simulink model "simulink"  (R2024b)
settings: Solver=ode15s  StartTime=0.0  StopTime=.3  RelTol=1e-3
values from neighbouring files (symbols this model uses):
  B_m = (kfi^2 * I_anl) / (V_an - R_a * I_anl)    (= 5.06615156069e-07)    [code.m]
  Jm = 5.05e-7    (= 5.05e-07)    [code.m]
  kfi = 9.18e-3    (= 0.00918)    [code.m]
  ki = 1/tc    (= 32.7207920792)    [code.m]
  kp = (tau_m+tau_e)/(tc+ tau_e)    (= 0.201485710943)    [code.m]
  L_a = 0.058e-3    (= 5.8e-05)    [code.m]
  R_a = 1.02    [code.m]
  ref_rpm = 10700    [code.m]
  T_n = 14.6e-3    (= 0.0146)    [code.m]
  tau_e = L_a / R_a    (= 5.6862745098e-05)    [code.m]
  tau_m = (Jm * R_a) / (kfi^2)    (= 0.0061123214718)    [code.m]
  V_an = 12    [code.m]
libraries: slpidlib x4, spsControlledVoltageSourceLib x2, spsDCMachineLib x2, sps_lib x1
settings Model: Creator=Compu City  LastModifiedBy=Compu City
settings SolverCC: MaxConsecutiveMinStep=5

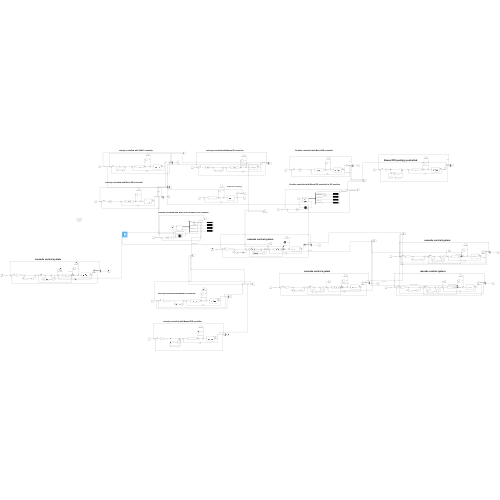
[thumbnail: Simulink's stored preview of the top-level diagram]
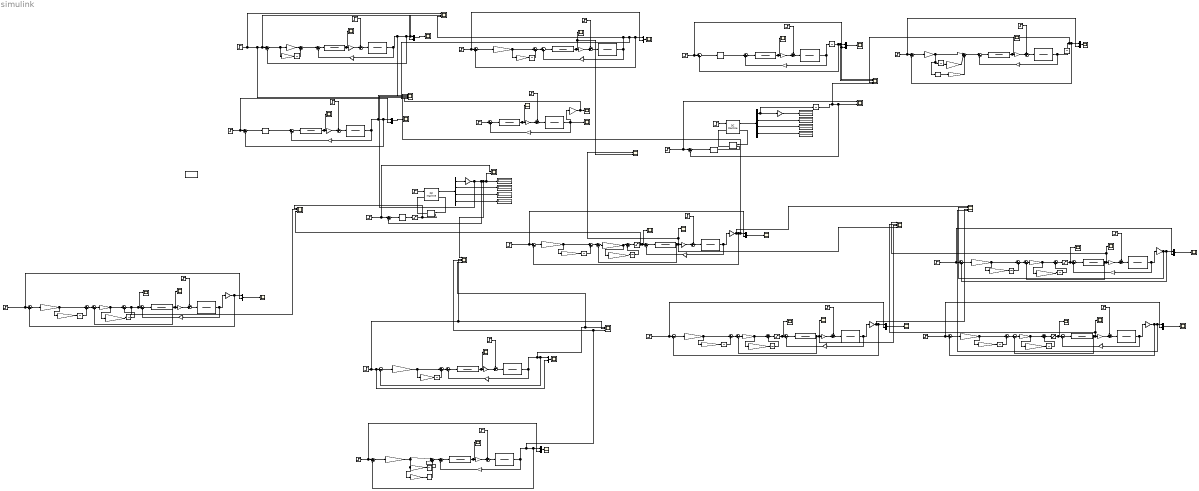
== system simulink ==
  note: Without Any controlling
  note: Manual PID position controlled
  note: velocity controlled with Manual PI controller
  note: velocity controlled with ICM PI controller
  note: velocity controlled with Block PID controller
  note: velocity controlled with Block PID controller in DC machine
  note: Position controlled with Block PID controller in DC machine
  note: Position controlled with Block PID controller
  note: cascade control system
  note: velocity controlled with Manual PI controller
  note: velocity controlled with Manual PID controller
  note: cascade control system
  note: cascade control system
  note: cascade control system
  note: cascade control system
  Bus Selector1 : BusSelector  OutputSignals=Speed wm (rad/s),Armature current ia (A),Field current if (A),Electrical torque Te (n m)
  Bus Selector2 : BusSelector  OutputSignals=Speed wm (rad/s),Armature current ia (A),Field current if (A),Electrical torque Te (n m)
  Controlled Voltage Source : spsControlledVoltageSourceLib/Controlled Voltage Source  Initialize=on  Source_Type=AC  Amplitude=0  Phase=0  Frequency=0  Measurements=None
  Controlled Voltage Source1 : spsControlledVoltageSourceLib/Controlled Voltage Source  Initialize=on  Source_Type=AC  Amplitude=0  Phase=0  Frequency=0  Measurements=None
  Current comparison : Scope  NumInputPorts=2
  DC permanent magnetic motor1 : spsDCMachineLib/DC Machine  PresetModel=No  MechanicalLoad=Torque TL  FieldType=Permanent magnet  ShowDetailedParameters=on  MeasurementBus=off  RLa=[1.02 5.8*10^-5]  RLf=[180 71.47]  Laf=1.345  MachineConstant=Torque constant (N.m/A)  Ke=1.8  Kt=kfi  J=Jm  Bm=B_m  Tf=0  w0=0  Ifinit=1  TsPowergui=0  TsBlock=-1
  DC permanent magnetic motor2 : spsDCMachineLib/DC Machine  PresetModel=No  MechanicalLoad=Torque TL  FieldType=Permanent magnet  ShowDetailedParameters=on  MeasurementBus=off  RLa=[1.02 5.8*10^-5]  RLf=[180 71.47]  Laf=1.345  MachineConstant=Torque constant (N.m/A)  Ke=1.8  Kt=kfi  J=Jm  Bm=B_m  Tf=0  w0=0  Ifinit=1  TsPowergui=0  TsBlock=-1
  Derivative : Derivative
  Derivative3 : Derivative
  Display{1..4,8..11} (8 alike) : Display
  External load{1..13} (13 alike) : Step  Time=0.02  After=T_n  SampleTime=0
  Gain : Gain  Gain=tau_e*60
  Gain1 : Gain  Gain=1/tau_m
  Gain{2,4..6,9..12,14..15,17..18,21,23,27..28,33,36..37,41..42,44,49..50,54..55} (26 alike) : Gain  Gain=kfi
  Gain{13,26,34..35,40,48} (6 alike) : Gain  Gain=1/(tau_m)
  Gain16 : Gain  Gain=30/pi
  Gain{8,19,45,51,56} (5 alike) : Gain  Gain=0.00705
  Gain20 : Gain  Gain=1/(tau_m*5)
  Gain22 : Gain  Gain=1/(tau_m/1000)
  Gain{24,47,53,58} (4 alike) : Gain  Gain=0.000705
  Gain25 : Gain  Gain=kp*10
  Gain29 : Gain  Gain=0.005
  Gain3 : Gain  Gain=ki
  Gain30 : Gain  Gain=1/(tau_m/1000)
  Gain31 : Gain  Gain=0.005
  Gain32 : Gain  Gain=1/(tau_m/10000)
  Gain38 : Gain  Gain=0.05
  Gain39 : Gain  Gain=tau_e
  Gain43 : Gain  Gain=0.05
  Gain46 : Gain  Gain=1/(tau_m/10000)
  Gain52 : Gain  Gain=1/(tau_m/10)
  Gain57 : Gain  Gain=1/(tau_m/1000)
  Gain7 : Gain  Gain=kp
  I{,1..5,8..9} (8 alike) : Scope
  Integrator{,1..17} (18 alike) : Integrator
  Mux{1..12} (12 alike) : Mux  Inputs=2
  PID Controller : slpidlib/PID Controller  Controller=PID  Form=Parallel  TimeDomain=Continuous-time  UseExternalTs=off  SampleTime=-1  IntegratorMethod=Forward Euler  FilterMethod=Forward Euler  ControllerParametersSource=internal  P=0.0119953669001722  I=2.21317544504697  UseKiTs=off  D=3.8924087618185e-06  UseExternalDerivativeSource=off  N=383.757391684538  UseFilter=on  TunerSelectOption=Transfer Function Based (PID Tuner App)  InitialConditionSource=internal  InitialConditionForIntegrator=0  InitialConditionForFilter=0  DifferentiatorICPrevScaledInput=0  ExternalReset=none  TrackingMode=off  Kt=1  LimitOutput=off  SatLimitsSource=internal  UpperSaturationLimit=inf  LowerSaturationLimit=-inf  LinearizeAsGain=on  AntiWindupMode=none  Kb=1  LimitIntegrator=off  UpperIntegratorSaturationLimit=inf  LowerIntegratorSaturationLimit=-inf  POutMin=[]  POutMax=[]  IOutMin=[]  IOutMax=[]  DOutMin=[]  DOutMax=[]  NOutMin=[]  NOutMax=[]  SumOutMin=[]  SumOutMax=[]  SaturationOutMin=[]  SaturationOutMax=[]  PParamMin=[]  PParamMax=[]  IParamMin=[]  IParamMax=[]  DParamMin=[]  DParamMax=[]  NParamMin=[]  NParamMax=[]  KbParamMin=[]  KbParamMax=[]  KtParamMin=[]  KtParamMax=[]  KbOutMin=[]  KbOutMax=[]  KtOutMin=[]  KtOutMax=[]  IntegratorOutMin=[]  IntegratorOutMax=[]  FilterOutMin=[]  FilterOutMax=[]  SumI1OutMin=[]  SumI1OutMax=[]  SumI2OutMin=[]  SumI2OutMax=[]  SumI3OutMin=[]  SumI3OutMax=[]  SumI4OutMin=[]  SumI4OutMax=[]  SumDOutMin=[]  SumDOutMax=[]  DifferentiatorOutMin=[]  DifferentiatorOutMax=[]  FilterDiffOutCoefMin=[]  FilterDiffOutCoefMax=[]  ReciprocalOutMin=[]  ReciprocalOutMax=[]  SumDenOutMin=[]  SumDenOutMax=[]  SumNumOutMin=[]  SumNumOutMax=[]  DivideOutMin=[]  DivideOutMax=[]  UdiffTsProdOutMin=[]  UdiffTsProdOutMax=[]  NTsProdOutMin=[]  NTsProdOutMax=[]  UintegralTsProdOutMin=[]  UintegralTsProdOutMax=[]  UngainTsProdOutMin=[]  UngainTsProdOutMax=[]  ClampingZeroOutDataTypeStr=Inherit: Inherit via back propagation  ClampingZeroOutMin=[]  ClampingZeroOutMax=[]  FilterDenConstantOutDataTypeStr=Inherit: Inherit via back propagation  FilterDenConstantOutMin=[]  FilterDenConstantOutMax=[]  PCopyOutDataTypeStr=Inherit: Inherit via back propagation  PCopyOutMin=[]  PCopyOutMax=[]  NCopyOutDataTypeStr=Inherit: Inherit via back propagation  NCopyOutMin=[]  NCopyOutMax=[]  IntegratorContinuousStateAttributes=''  IntegratorStateMustResolveToSignalObject=off  IntegratorRTWStateStorageClass=Auto  FilterContinuousStateAttributes=''  FilterStateMustResolveToSignalObject=off  FilterRTWStateStorageClass=Auto  ParallelPVariant=InternalParameters  IdealPVariant=Disabled  IVariant=InternalParameters  DVariant=InternalParameters  IntegratorVariant=Continuous  SatVariant=Disabled  AWVariant=Passthrough  PCopyVariant=Disabled  TRVariant=Disabled  FdbkBlocksVariant=Forward  IdealPFdbkVariant=Disabled  SatFdbkVariant=Disabled  DerivativeFilterVariant=ContFilter  NVariant=InternalParameters  NCopyVariant=Disabled  FilterICVariant=InternalICsFilter  IntegratorICVariant=InternalICs  ExternalResetVariant=Disabled  TRSumVariant=Passthrough  SumFdbkVariant=Disabled  SumVariant=Sum_PID  TsampFilterVariant=InternalTs  TsampNgainVariant=Passthrough  TsampIntegralVariant=Disabled_SignalSpec  ExternalSaturationOutDataTypeStr=Inherit: Same as second input  DerivativeSourceVariant=ErrorSignal  PreIntVariant=InternalPreInt
  PID Controller1 : slpidlib/PID Controller  Controller=PID  Form=Parallel  TimeDomain=Continuous-time  UseExternalTs=off  SampleTime=-1  IntegratorMethod=Forward Euler  FilterMethod=Forward Euler  ControllerParametersSource=internal  P=0.00135864322894718  I=0.306131273508745  UseKiTs=off  D=4.02045915696409e-07  UseExternalDerivativeSource=off  N=693.137788969892  UseFilter=on  TunerSelectOption=Transfer Function Based (PID Tuner App)  InitialConditionSource=internal  InitialConditionForIntegrator=0  InitialConditionForFilter=0  DifferentiatorICPrevScaledInput=0  ExternalReset=none  TrackingMode=off  Kt=1  LimitOutput=off  SatLimitsSource=internal  UpperSaturationLimit=inf  LowerSaturationLimit=-inf  LinearizeAsGain=on  AntiWindupMode=none  Kb=1  LimitIntegrator=off  UpperIntegratorSaturationLimit=inf  LowerIntegratorSaturationLimit=-inf  POutMin=[]  POutMax=[]  IOutMin=[]  IOutMax=[]  DOutMin=[]  DOutMax=[]  NOutMin=[]  NOutMax=[]  SumOutMin=[]  SumOutMax=[]  SaturationOutMin=[]  SaturationOutMax=[]  PParamMin=[]  PParamMax=[]  IParamMin=[]  IParamMax=[]  DParamMin=[]  DParamMax=[]  NParamMin=[]  NParamMax=[]  KbParamMin=[]  KbParamMax=[]  KtParamMin=[]  KtParamMax=[]  KbOutMin=[]  KbOutMax=[]  KtOutMin=[]  KtOutMax=[]  IntegratorOutMin=[]  IntegratorOutMax=[]  FilterOutMin=[]  FilterOutMax=[]  SumI1OutMin=[]  SumI1OutMax=[]  SumI2OutMin=[]  SumI2OutMax=[]  SumI3OutMin=[]  SumI3OutMax=[]  SumI4OutMin=[]  SumI4OutMax=[]  SumDOutMin=[]  SumDOutMax=[]  DifferentiatorOutMin=[]  DifferentiatorOutMax=[]  FilterDiffOutCoefMin=[]  FilterDiffOutCoefMax=[]  ReciprocalOutMin=[]  ReciprocalOutMax=[]  SumDenOutMin=[]  SumDenOutMax=[]  SumNumOutMin=[]  SumNumOutMax=[]  DivideOutMin=[]  DivideOutMax=[]  UdiffTsProdOutMin=[]  UdiffTsProdOutMax=[]  NTsProdOutMin=[]  NTsProdOutMax=[]  UintegralTsProdOutMin=[]  UintegralTsProdOutMax=[]  UngainTsProdOutMin=[]  UngainTsProdOutMax=[]  ClampingZeroOutDataTypeStr=Inherit: Inherit via back propagation  ClampingZeroOutMin=[]  ClampingZeroOutMax=[]  FilterDenConstantOutDataTypeStr=Inherit: Inherit via back propagation  FilterDenConstantOutMin=[]  FilterDenConstantOutMax=[]  PCopyOutDataTypeStr=Inherit: Inherit via back propagation  PCopyOutMin=[]  PCopyOutMax=[]  NCopyOutDataTypeStr=Inherit: Inherit via back propagation  NCopyOutMin=[]  NCopyOutMax=[]  IntegratorContinuousStateAttributes=''  IntegratorStateMustResolveToSignalObject=off  IntegratorRTWStateStorageClass=Auto  FilterContinuousStateAttributes=''  FilterStateMustResolveToSignalObject=off  FilterRTWStateStorageClass=Auto  ParallelPVariant=InternalParameters  IdealPVariant=Disabled  IVariant=InternalParameters  DVariant=InternalParameters  IntegratorVariant=Continuous  SatVariant=Disabled  AWVariant=Passthrough  PCopyVariant=Disabled  TRVariant=Disabled  FdbkBlocksVariant=Forward  IdealPFdbkVariant=Disabled  SatFdbkVariant=Disabled  DerivativeFilterVariant=ContFilter  NVariant=InternalParameters  NCopyVariant=Disabled  FilterICVariant=InternalICsFilter  IntegratorICVariant=InternalICs  ExternalResetVariant=Disabled  TRSumVariant=Passthrough  SumFdbkVariant=Disabled  SumVariant=Sum_PID  TsampFilterVariant=InternalTs  TsampNgainVariant=Passthrough  TsampIntegralVariant=Disabled_SignalSpec  ExternalSaturationOutDataTypeStr=Inherit: Same as second input  DerivativeSourceVariant=ErrorSignal  PreIntVariant=InternalPreInt
  PID Controller2 : slpidlib/PID Controller  Controller=PID  Form=Parallel  TimeDomain=Continuous-time  UseExternalTs=off  SampleTime=-1  IntegratorMethod=Forward Euler  FilterMethod=Forward Euler  ControllerParametersSource=internal  P=8.0055285463139  I=469.188134848807  UseKiTs=off  D=0.034037625993495  UseExternalDerivativeSource=off  N=70209.7443182031  UseFilter=on  TunerSelectOption=Transfer Function Based (PID Tuner App)  InitialConditionSource=internal  InitialConditionForIntegrator=0  InitialConditionForFilter=0  DifferentiatorICPrevScaledInput=0  ExternalReset=none  TrackingMode=off  Kt=1  LimitOutput=off  SatLimitsSource=internal  UpperSaturationLimit=inf  LowerSaturationLimit=-inf  LinearizeAsGain=on  AntiWindupMode=none  Kb=1  LimitIntegrator=off  UpperIntegratorSaturationLimit=inf  LowerIntegratorSaturationLimit=-inf  POutMin=[]  POutMax=[]  IOutMin=[]  IOutMax=[]  DOutMin=[]  DOutMax=[]  NOutMin=[]  NOutMax=[]  SumOutMin=[]  SumOutMax=[]  SaturationOutMin=[]  SaturationOutMax=[]  PParamMin=[]  PParamMax=[]  IParamMin=[]  IParamMax=[]  DParamMin=[]  DParamMax=[]  NParamMin=[]  NParamMax=[]  KbParamMin=[]  KbParamMax=[]  KtParamMin=[]  KtParamMax=[]  KbOutMin=[]  KbOutMax=[]  KtOutMin=[]  KtOutMax=[]  IntegratorOutMin=[]  IntegratorOutMax=[]  FilterOutMin=[]  FilterOutMax=[]  SumI1OutMin=[]  SumI1OutMax=[]  SumI2OutMin=[]  SumI2OutMax=[]  SumI3OutMin=[]  SumI3OutMax=[]  SumI4OutMin=[]  SumI4OutMax=[]  SumDOutMin=[]  SumDOutMax=[]  DifferentiatorOutMin=[]  DifferentiatorOutMax=[]  FilterDiffOutCoefMin=[]  FilterDiffOutCoefMax=[]  ReciprocalOutMin=[]  ReciprocalOutMax=[]  SumDenOutMin=[]  SumDenOutMax=[]  SumNumOutMin=[]  SumNumOutMax=[]  DivideOutMin=[]  DivideOutMax=[]  UdiffTsProdOutMin=[]  UdiffTsProdOutMax=[]  NTsProdOutMin=[]  NTsProdOutMax=[]  UintegralTsProdOutMin=[]  UintegralTsProdOutMax=[]  UngainTsProdOutMin=[]  UngainTsProdOutMax=[]  ClampingZeroOutDataTypeStr=Inherit: Inherit via back propagation  ClampingZeroOutMin=[]  ClampingZeroOutMax=[]  FilterDenConstantOutDataTypeStr=Inherit: Inherit via back propagation  FilterDenConstantOutMin=[]  FilterDenConstantOutMax=[]  PCopyOutDataTypeStr=Inherit: Inherit via back propagation  PCopyOutMin=[]  PCopyOutMax=[]  NCopyOutDataTypeStr=Inherit: Inherit via back propagation  NCopyOutMin=[]  NCopyOutMax=[]  IntegratorContinuousStateAttributes=''  IntegratorStateMustResolveToSignalObject=off  IntegratorRTWStateStorageClass=Auto  FilterContinuousStateAttributes=''  FilterStateMustResolveToSignalObject=off  FilterRTWStateStorageClass=Auto  ParallelPVariant=InternalParameters  IdealPVariant=Disabled  IVariant=InternalParameters  DVariant=InternalParameters  IntegratorVariant=Continuous  SatVariant=Disabled  AWVariant=Passthrough  PCopyVariant=Disabled  TRVariant=Disabled  FdbkBlocksVariant=Forward  IdealPFdbkVariant=Disabled  SatFdbkVariant=Disabled  DerivativeFilterVariant=ContFilter  NVariant=InternalParameters  NCopyVariant=Disabled  FilterICVariant=InternalICsFilter  IntegratorICVariant=InternalICs  ExternalResetVariant=Disabled  TRSumVariant=Passthrough  SumFdbkVariant=Disabled  SumVariant=Sum_PID  TsampFilterVariant=InternalTs  TsampNgainVariant=Passthrough  TsampIntegralVariant=Disabled_SignalSpec  ExternalSaturationOutDataTypeStr=Inherit: Same as second input  DerivativeSourceVariant=ErrorSignal  PreIntVariant=InternalPreInt
  PID Controller3 : slpidlib/PID Controller  Controller=PID  Form=Parallel  TimeDomain=Continuous-time  UseExternalTs=off  SampleTime=-1  IntegratorMethod=Forward Euler  FilterMethod=Forward Euler  ControllerParametersSource=internal  P=16.6827824255638  I=704.189736175567  UseKiTs=off  D=0.0978151293443874  UseExternalDerivativeSource=off  N=92341.2012278854  UseFilter=on  TunerSelectOption=Transfer Function Based (PID Tuner App)  InitialConditionSource=internal  InitialConditionForIntegrator=0  InitialConditionForFilter=0  DifferentiatorICPrevScaledInput=0  ExternalReset=none  TrackingMode=off  Kt=1  LimitOutput=off  SatLimitsSource=internal  UpperSaturationLimit=inf  LowerSaturationLimit=-inf  LinearizeAsGain=on  AntiWindupMode=none  Kb=1  LimitIntegrator=off  UpperIntegratorSaturationLimit=inf  LowerIntegratorSaturationLimit=-inf  POutMin=[]  POutMax=[]  IOutMin=[]  IOutMax=[]  DOutMin=[]  DOutMax=[]  NOutMin=[]  NOutMax=[]  SumOutMin=[]  SumOutMax=[]  SaturationOutMin=[]  SaturationOutMax=[]  PParamMin=[]  PParamMax=[]  IParamMin=[]  IParamMax=[]  DParamMin=[]  DParamMax=[]  NParamMin=[]  NParamMax=[]  KbParamMin=[]  KbParamMax=[]  KtParamMin=[]  KtParamMax=[]  KbOutMin=[]  KbOutMax=[]  KtOutMin=[]  KtOutMax=[]  IntegratorOutMin=[]  IntegratorOutMax=[]  FilterOutMin=[]  FilterOutMax=[]  SumI1OutMin=[]  SumI1OutMax=[]  SumI2OutMin=[]  SumI2OutMax=[]  SumI3OutMin=[]  SumI3OutMax=[]  SumI4OutMin=[]  SumI4OutMax=[]  SumDOutMin=[]  SumDOutMax=[]  DifferentiatorOutMin=[]  DifferentiatorOutMax=[]  FilterDiffOutCoefMin=[]  FilterDiffOutCoefMax=[]  ReciprocalOutMin=[]  ReciprocalOutMax=[]  SumDenOutMin=[]  SumDenOutMax=[]  SumNumOutMin=[]  SumNumOutMax=[]  DivideOutMin=[]  DivideOutMax=[]  UdiffTsProdOutMin=[]  UdiffTsProdOutMax=[]  NTsProdOutMin=[]  NTsProdOutMax=[]  UintegralTsProdOutMin=[]  UintegralTsProdOutMax=[]  UngainTsProdOutMin=[]  UngainTsProdOutMax=[]  ClampingZeroOutDataTypeStr=Inherit: Inherit via back propagation  ClampingZeroOutMin=[]  ClampingZeroOutMax=[]  FilterDenConstantOutDataTypeStr=Inherit: Inherit via back propagation  FilterDenConstantOutMin=[]  FilterDenConstantOutMax=[]  PCopyOutDataTypeStr=Inherit: Inherit via back propagation  PCopyOutMin=[]  PCopyOutMax=[]  NCopyOutDataTypeStr=Inherit: Inherit via back propagation  NCopyOutMin=[]  NCopyOutMax=[]  IntegratorContinuousStateAttributes=''  IntegratorStateMustResolveToSignalObject=off  IntegratorRTWStateStorageClass=Auto  FilterContinuousStateAttributes=''  FilterStateMustResolveToSignalObject=off  FilterRTWStateStorageClass=Auto  ParallelPVariant=InternalParameters  IdealPVariant=Disabled  IVariant=InternalParameters  DVariant=InternalParameters  IntegratorVariant=Continuous  SatVariant=Disabled  AWVariant=Passthrough  PCopyVariant=Disabled  TRVariant=Disabled  FdbkBlocksVariant=Forward  IdealPFdbkVariant=Disabled  SatFdbkVariant=Disabled  DerivativeFilterVariant=ContFilter  NVariant=InternalParameters  NCopyVariant=Disabled  FilterICVariant=InternalICsFilter  IntegratorICVariant=InternalICs  ExternalResetVariant=Disabled  TRSumVariant=Passthrough  SumFdbkVariant=Disabled  SumVariant=Sum_PID  TsampFilterVariant=InternalTs  TsampNgainVariant=Passthrough  TsampIntegralVariant=Disabled_SignalSpec  ExternalSaturationOutDataTypeStr=Inherit: Same as second input  DerivativeSourceVariant=ErrorSignal  PreIntVariant=InternalPreInt
  Saturation{1..3,5..6} (5 alike) : Saturate  UpperLimit=V_an  LowerLimit=-V_an
  Scope{,5,7,9..10} (5 alike) : Scope
  Scope1 : Scope  NumInputPorts=3
  Scope11 : Scope  NumInputPorts=3
  Scope{6,8,12,14} (4 alike) : Scope  NumInputPorts=4
  Scope13 : Scope  NumInputPorts=3
  Scope2 : Scope  NumInputPorts=2
  Scope3 : Scope  NumInputPorts=7
  Scope4 : Scope  NumInputPorts=2
  Sum{,1..2,5,7..9,11,13,16..18,21..23,27..28,31..32,34,37..38,41..42,45..46,48,51..52,54,57..58} (32 alike) : Sum  Inputs=|+-
  Sum{3,10,12,14..15,19,25,29,35,39,43,49,55} (13 alike) : Sum  Inputs=-+|
  Sum{4,6,20,24,30,33,36,44,47,50,53,56,59} (13 alike) : Sum  Inputs=|++
  Sum26 : Sum  Inputs=|+++
  Sum40 : Sum  Inputs=|+++
  T_N : Step  Time=0.02  After=T_n  SampleTime=0
  T_N1 : Step  Time=0.02  After=T_n  SampleTime=0
  Transfer Fcn{1..2,5,7,9,11,13,15,17,19,21,23,25} (13 alike) : TransferFcn  Denominator=[ L_a R_a]
  Transfer Fcn{3..4,6,8,10,12,14,16,18,20,22,24,26} (13 alike) : TransferFcn  Denominator=[ Jm B_m ]
  U(S){1..2,4,6,8..13} (10 alike) : Step  Time=0.02  After=ref_rpm  SampleTime=0
  U(S)3 : Step  Time=0.02  After=V_an  SampleTime=0
  U(S)5 : Step  Time=0.02  After=pi  SampleTime=0
  U(S)7 : Step  Time=0.02  After=pi  SampleTime=0
  U(t)1 : Step  Time=0.02  After=pi  SampleTime=0
  U(t)2 : Step  Time=0.02  After=ref_rpm  SampleTime=0
  current{,1..4} (5 alike) : Scope
  powergui : sps_lib/powergui  Priority=1  SimulationMode=Continuous  SampleTime=50e-6  frequency=60  Iterations=50  frequencyindice=0  Pbase=100e6  ErrMax=1e-4  UnitsV=kV  UnitsW=MW  buscounter=0  FunctionMessages=off  echomessages=off  EnableUseOfTLC=off  CurrentSourceSwitches=off  DisableSnubberDevices=off  DisableRonSwitches=off  DisableVfSwitches=off  DisplayEquations=off  AutomaticDiscreteSolvers=off  SolverType=Tustin/Backward Euler (TBE)  Interpol=off  ExternalGateDelay=off  methode=off  Ts=100  x0status=blocks  SPID=on  SwTol=0  HookPort=off  NonlinearTolerance=1e-4  nMaxIteration=100  ContinueOnMaxIteration=off  RestoreLinks=warning  ResistiveCurrentMeasurement=off  Frange=[0:2:500]  Ylog=off  Xlog=on  ShowGrid=off  save=off  variable=ZData  structure=0  ZoomFFT=off  StartTime=0.0  cycles=1  DisplayStyle=1  fundamental=60  FreqAxis=off  MaxFrequency=1000  frequencyindicesteady=1  RmsSteady=1  display=off
  rad/s2rpm{1..7} (7 alike) : Gain  Gain=30/pi
  rad/s4 : Scope
  rpm{1..8} (8 alike) : Scope
  voltage{,1..4} (5 alike) : Scope
  wires:
  Gain1/1 -> Integrator1/1
  External load2/1 -> Sum10/1  "T-load"
  Gain8/1 -> Gain1/1, Sum4/1
  Sum1/1 -> Gain8/1
  Transfer Fcn1/1 -> Current comparison/2, I/1, Gain2/1  "Single loop  current"
  U(S)2/1 -> Mux1/2, Sum1/1
  Sum4/1 -> Sum5/1
  Transfer Fcn4/1 -> Gain6/1, Scope3/7, Mux1/1, Sum1/2, Scope1/3  "PI controller"
  Integrator1/1 -> Sum4/2
  Gain6/1 -> Sum5/2
  Sum10/1 -> Transfer Fcn4/1
  Gain2/1 -> Sum10/2
  Sum5/1 -> Transfer Fcn1/1
  Mux1/1 -> Scope/1
  Gain3/1 -> Integrator2/1
  External load1/1 -> Sum3/1  "T-load"
  Gain7/1 -> Sum6/1
  Sum2/1 -> Gain3/1, Gain7/1
  Transfer Fcn2/1 -> I1/1, Gain4/1  "i-a"
  U(S)1/1 -> Scope1/1, Scope3/5, Mux2/2, Sum2/1  "refrence"
  Mux2/1 -> rpm2/1
  Integrator2/1 -> Sum6/2
  Gain5/1 -> Sum7/2
  Sum3/1 -> Transfer Fcn3/1
  Gain4/1 -> Sum3/2
  Transfer Fcn3/1 -> Gain5/1, Scope3/2, Sum2/2, Scope1/2, Mux2/1  "PI using ICM"
  Sum7/1 -> Transfer Fcn2/1
  Sum14/1 -> Transfer Fcn8/1
  Gain15/1 -> Sum16/2
  External load4/1 -> Sum14/1  "T-load"
  Transfer Fcn8/1 -> Gain15/1, Scope3/3, Sum13/2, Mux4/1  "PID block"
  U(S)4/1 -> Mux4/2, Sum13/1
  Transfer Fcn7/1 -> I4/1, Gain14/1  "i-a"
  Mux4/1 -> rpm1/1
  Sum16/1 -> Transfer Fcn7/1
  Gain14/1 -> Sum14/2
  Sum13/1 -> PID Controller/1
  Gain10/1 -> Sum11/2
  External load3/1 -> Sum12/1  "T-load"
  Gain9/1 -> Sum12/2
  Sum12/1 -> Transfer Fcn6/1
  Transfer Fcn5/1 -> I3/1, Gain9/1  "i-a"
  U(S)3/1 -> Sum11/1
  Gain16/1 -> Scope3/6, rpm4/1  "UNcontrolled"
  Transfer Fcn6/1 -> Gain10/1, Gain16/1, rad/s4/1
  Sum11/1 -> Transfer Fcn5/1
  Sum/1 -> PID Controller1/1
  Bus Selector2/1 -> rad/s2rpm2/1  "<Speed wm (rad/s)>"
  Bus Selector2/3 -> Display10/1  "<Field current if (A)>"
  DC permanent magnetic motor2/1 -> Bus Selector2/1
  Bus Selector2/2 -> Display9/1  "<Armature current ia (A)>"
  Bus Selector2/4 -> Display11/1  "<Electrical torque Te (n m)>"
  rad/s2rpm2/1 -> Scope3/4, Sum/2, Scope8/1, Scope2/2, Display8/1  "DC machine PID"
  U(t)2/1 -> Sum/1, Scope2/1  "Refrence"
  T_N/1 -> DC permanent magnetic motor2/1
  PID Controller2/1 -> Controlled Voltage Source1/1
  T_N1/1 -> DC permanent magnetic motor1/1
  DC permanent magnetic motor1/1 -> Bus Selector1/1
  Bus Selector1/4 -> Display2/1  "<Electrical torque Te (n m)>"
  Bus Selector1/2 -> Display4/1  "<Armature current ia (A)>"
  rad/s2rpm1/1 -> Display3/1
  U(t)1/1 -> Sum8/1, Scope4/1  "Refrence"
  Bus Selector1/1 -> Integrator/1, rad/s2rpm1/1  "<Speed wm (rad/s)>"
  Bus Selector1/3 -> Display1/1  "<Field current if (A)>"
  Sum8/1 -> PID Controller2/1
  Integrator/1 -> Scope6/4, Sum8/2, Scope4/2  "Position DC machine"
  U(S)5/1 -> Scope6/1, Mux3/2, Sum9/1  "refrence"
  Gain11/1 -> Sum15/2
  Transfer Fcn9/1 -> I5/1, Gain11/1  "i-a"
  Sum17/1 -> Transfer Fcn9/1
  Transfer Fcn10/1 -> Gain12/1, Integrator3/1
  External load5/1 -> Sum15/1  "T-load"
  Sum15/1 -> Transfer Fcn10/1
  Gain12/1 -> Sum17/2
  Sum9/1 -> PID Controller3/1
  PID Controller3/1 -> Sum17/1
  Integrator3/1 -> Sum9/2, Scope6/2, Mux3/1  "Position PID block"
  Mux3/1 -> Scope5/1
  Sum19/1 -> Transfer Fcn12/1
  Gain18/1 -> Sum21/2
  External load6/1 -> Sum19/1  "T-load"
  Transfer Fcn12/1 -> Gain18/1, rad/s2rpm3/1
  U(S)6/1 -> Mux5/2, Sum18/1  "refrence"
  Transfer Fcn11/1 -> current/1, Current comparison/1, Scope12/4, Gain17/1, Sum22/2  "Cascade current"
  Mux5/1 -> rpm3/1
  Sum21/1 -> Transfer Fcn11/1
  Gain17/1 -> Sum19/2
  Sum20/1 -> Sum22/1
  Integrator4/1 -> Sum20/2
  Gain13/1 -> Integrator4/1
  Sum18/1 -> Gain19/1
  Gain19/1 -> Sum20/1, Gain13/1
  Gain24/1 -> Sum24/1, Gain22/1
  Integrator6/1 -> Sum24/2
  Gain22/1 -> Integrator6/1
  Sum22/1 -> Gain24/1
  Sum24/1 -> Saturation1/1
  rad/s2rpm3/1 -> Scope3/1, Mux5/1, Sum18/2, Scope14/1  "RPM Cascade"
  Saturation1/1 -> Scope13/3, voltage/1, Sum21/1  "cascade with saturation"
  External load7/1 -> Sum25/1  "T-load"
  Gain21/1 -> Sum25/2
  Gain23/1 -> Sum27/2
  Sum27/1 -> Transfer Fcn13/1
  Sum25/1 -> Transfer Fcn14/1
  Transfer Fcn13/1 -> I2/1, Gain21/1  "Single loop  current"
  Integrator5/1 -> Gain20/1
  Sum23/1 -> Gain25/1
  Transfer Fcn14/1 -> Gain23/1, Integrator7/1  "PI controller"
  U(S)7/1 -> Mux6/2, Sum23/1  "refrence"
  Mux6/1 -> Scope7/1
  Integrator7/1 -> Scope6/3, Mux6/1, Sum23/2  "Manual PID position"
  Sum34/1 -> Gain38/1
  Transfer Fcn20/1 -> Scope8/4, Scope11/1, Mux8/1, Sum34/2, Gain37/1  "PI controller2"
  Mux8/1 -> Scope9/1
  Gain37/1 -> Sum37/2
  U(S)10/1 -> Scope11/2, Scope8/2, Mux8/2, Sum34/1
  External load10/1 -> Sum35/1  "T-load"
  Integrator9/1 -> Sum36/2
  Transfer Fcn19/1 -> I8/1, Gain36/1  "Single loop  current"
  Gain35/1 -> Integrator9/1
  Sum35/1 -> Transfer Fcn20/1
  Sum37/1 -> Transfer Fcn19/1
  Gain38/1 -> Gain35/1, Sum36/1
  Gain36/1 -> Sum35/2
  Sum38/1 -> Gain43/1
  Transfer Fcn22/1 -> Scope8/3, Scope11/3, Mux9/1, Sum38/2, Gain42/1  "PID controller3"
  Mux9/1 -> Scope10/1
  Gain42/1 -> Sum41/2
  U(S)11/1 -> Mux9/2, Sum38/1
  External load11/1 -> Sum39/1  "T-load"
  Derivative3/1 -> Sum40/3
  Gain39/1 -> Derivative3/1
  Sum40/1 -> Sum41/1
  Integrator10/1 -> Sum40/2
  Transfer Fcn21/1 -> I9/1, Gain41/1  "Single loop  current"
  Gain40/1 -> Integrator10/1
  Sum39/1 -> Transfer Fcn22/1
  Sum41/1 -> Transfer Fcn21/1
  Gain43/1 -> Gain39/1, Gain40/1, Sum40/1
  Gain41/1 -> Sum39/2
  PID Controller1/1 -> Saturation3/1
  Gain25/1 -> Derivative/1, Integrator5/1, Sum26/1
  Gain20/1 -> Sum26/2
  Derivative/1 -> Gain/1
  Gain/1 -> Sum26/3
  Sum26/1 -> Sum27/1
  Saturation3/1 -> Scope13/1, Controlled Voltage Source/1  "DC mahcine with saturation"
  Sum6/1 -> Sum7/1
  Sum36/1 -> Sum37/1
  PID Controller/1 -> Sum16/1
  rad/s2rpm4/1 -> Scope14/2, Mux7/1, Sum28/2  "RPM lower p"
  Transfer Fcn15/1 -> Scope12/1, current1/1, Gain27/1, Sum32/2  "Cascade current lower P"
  Sum31/1 -> Transfer Fcn15/1
  Gain27/1 -> Sum29/2
  Gain28/1 -> Sum31/2
  Sum32/1 -> Gain31/1
  Integrator11/1 -> Sum33/2
  Transfer Fcn16/1 -> Gain28/1, rad/s2rpm4/1  "PI block"
  U(S)8/1 -> Mux7/2, Sum28/1  "refrence"
  Gain26/1 -> Integrator8/1
  Gain31/1 -> Gain30/1, Sum33/1
  External load8/1 -> Sum29/1  "T-load"
  Sum33/1 -> Saturation2/1
  Sum29/1 -> Transfer Fcn16/1
  Sum28/1 -> Gain29/1
  Gain29/1 -> Sum30/1, Gain26/1
  Saturation2/1 -> voltage1/1, Sum31/1
  Integrator8/1 -> Sum30/2
  Gain30/1 -> Integrator11/1
  Mux7/1 -> rpm5/1
  Sum30/1 -> Sum32/1
  Sum46/1 -> Gain47/1
  Gain44/1 -> Sum45/2
  Transfer Fcn17/1 -> current2/1, Scope12/3, Gain33/1, Sum46/2  "Cascade current lower tau"
  Sum45/1 -> Transfer Fcn17/1
  Integrator12/1 -> Sum47/2
  Sum44/1 -> Sum46/1
  Gain46/1 -> Integrator12/1
  Sum43/1 -> Transfer Fcn18/1
  Gain33/1 -> Sum43/2
  Mux10/1 -> rpm6/1
  Sum47/1 -> Saturation5/1
  Integrator13/1 -> Sum44/2
  Gain45/1 -> Sum44/1, Gain32/1
  Saturation5/1 -> voltage2/1, Sum45/1
  rad/s2rpm5/1 -> Scope14/3, Mux10/1, Sum42/2  "With lower tau"
  Gain32/1 -> Integrator13/1
  External load9/1 -> Sum43/1  "T-load"
  U(S)9/1 -> Mux10/2, Sum42/1  "refrence"
  Sum42/1 -> Gain45/1
  Transfer Fcn18/1 -> Gain44/1, rad/s2rpm5/1  "PI block"
  Gain47/1 -> Gain46/1, Sum47/1
  Sum52/1 -> Gain53/1
  Gain50/1 -> Sum51/2
  Transfer Fcn23/1 -> current3/1, Scope12/2, Gain49/1, Sum52/2  "Cascade current with higher tau m"
  Sum51/1 -> Transfer Fcn23/1
  Integrator14/1 -> Sum53/2
  Sum50/1 -> Sum52/1
  Gain52/1 -> Integrator14/1
  Sum49/1 -> Transfer Fcn24/1
  Gain49/1 -> Sum49/2
  Mux11/1 -> rpm7/1
  Sum53/1 -> Saturation6/1
  Integrator15/1 -> Sum50/2
  Gain51/1 -> Sum50/1, Gain48/1
  Saturation6/1 -> voltage3/1, Sum51/1
  rad/s2rpm6/1 -> Scope14/4, Mux11/1, Sum48/2  "with higher Tau"
  Gain48/1 -> Integrator15/1
  External load12/1 -> Sum49/1  "T-load"
  U(S)12/1 -> Mux11/2, Sum48/1  "refrence"
  Sum48/1 -> Gain51/1
  Transfer Fcn24/1 -> Gain50/1, rad/s2rpm6/1  "PI block"
  Gain53/1 -> Gain52/1, Sum53/1
  rad/s2rpm7/1 -> Mux12/1, Sum54/2  "RPM Cascade"
  Transfer Fcn25/1 -> current4/1, Gain54/1, Sum58/2  "Cascade current"
  Sum57/1 -> Transfer Fcn25/1
  Gain54/1 -> Sum55/2
  Gain55/1 -> Sum57/2
  Sum58/1 -> Gain58/1
  Integrator17/1 -> Sum59/2
  Transfer Fcn26/1 -> Gain55/1, rad/s2rpm7/1  "PI block"
  U(S)13/1 -> Mux12/2, Sum54/1  "refrence"
  Gain34/1 -> Integrator16/1
  Gain58/1 -> Gain57/1, Sum59/1
  External load13/1 -> Sum55/1  "T-load"
  Sum55/1 -> Transfer Fcn26/1
  Sum54/1 -> Gain56/1
  Gain56/1 -> Sum56/1, Gain34/1
  Sum59/1 -> Scope13/2, voltage4/1, Sum57/1  "without saturation"
  Integrator16/1 -> Sum56/2
  Gain57/1 -> Integrator17/1
  Mux12/1 -> rpm8/1
  Sum56/1 -> Sum58/1
  connections:
  Controlled Voltage Source/RConn1 -- DC permanent magnetic motor2/LConn1
  Controlled Voltage Source/LConn1 -- DC permanent magnetic motor2/RConn1
  Controlled Voltage Source1/RConn1 -- DC permanent magnetic motor1/LConn1
  Controlled Voltage Source1/LConn1 -- DC permanent magnetic motor1/RConn1
